simulink model "rfsoc4x2_ospfb_128"  (R2021a)
settings: Solver=VariableStepAuto  StartTime=0.0  StopTime=2048  RelTol=1e-3
undefined symbols (not defined in the file): pfb_coeff_gen_calc
libraries: xbsIndex_r4 x37092, casper_library_delays x737, casper_library_misc x68, xps_library x1
(part 146 of 339)

== system rfsoc4x2_ospfb_128/fft2/fft_unscrambler/debus4 ==
  bus_in : Inport
  reinterpret1 : xbsIndex_r4/Reinterpret  force_arith_type=on  arith_type=Unsigned  force_bin_pt=on  bin_pt=0  block_type=reinterpret
  slice1 : xbsIndex_r4/Slice  nbits=36  boolean_output=off  mode=Upper Bit Location + Width  bit1=0  base1=MSB of Input  bit0=0  base0=LSB of Input  dbl_ovrd=off  block_type=slice
  msb_lsb_out1 : Outport
  wires:
  reinterpret1/1 -> msb_lsb_out1/1
  slice1/1 -> reinterpret1/1
  bus_in/1 -> slice1/1

== system rfsoc4x2_ospfb_128/fft2/fft_unscrambler/debus5 ==
  bus_in : Inport
  reinterpret1 : xbsIndex_r4/Reinterpret  force_arith_type=on  arith_type=Unsigned  force_bin_pt=on  bin_pt=0  block_type=reinterpret
  slice1 : xbsIndex_r4/Slice  nbits=36  boolean_output=off  mode=Upper Bit Location + Width  bit1=0  base1=MSB of Input  bit0=0  base0=LSB of Input  dbl_ovrd=off  block_type=slice
  msb_lsb_out1 : Outport
  wires:
  reinterpret1/1 -> msb_lsb_out1/1
  slice1/1 -> reinterpret1/1
  bus_in/1 -> slice1/1

== system rfsoc4x2_ospfb_128/fft2/fft_unscrambler/debus6 ==
  bus_in : Inport
  reinterpret1 : xbsIndex_r4/Reinterpret  force_arith_type=on  arith_type=Unsigned  force_bin_pt=on  bin_pt=0  block_type=reinterpret
  slice1 : xbsIndex_r4/Slice  nbits=36  boolean_output=off  mode=Upper Bit Location + Width  bit1=0  base1=MSB of Input  bit0=0  base0=LSB of Input  dbl_ovrd=off  block_type=slice
  msb_lsb_out1 : Outport
  wires:
  reinterpret1/1 -> msb_lsb_out1/1
  slice1/1 -> reinterpret1/1
  bus_in/1 -> slice1/1

== system rfsoc4x2_ospfb_128/fft2/fft_unscrambler/debus7 ==
  bus_in : Inport
  reinterpret1 : xbsIndex_r4/Reinterpret  force_arith_type=on  arith_type=Unsigned  force_bin_pt=on  bin_pt=0  block_type=reinterpret
  slice1 : xbsIndex_r4/Slice  nbits=36  boolean_output=off  mode=Upper Bit Location + Width  bit1=0  base1=MSB of Input  bit0=0  base0=LSB of Input  dbl_ovrd=off  block_type=slice
  msb_lsb_out1 : Outport
  wires:
  reinterpret1/1 -> msb_lsb_out1/1
  slice1/1 -> reinterpret1/1
  bus_in/1 -> slice1/1

== system rfsoc4x2_ospfb_128/fft2/fft_unscrambler/reorder ==
  sync : Inport
  en : Inport  Port=2
  din0 : Inport  Port=3
  din1 : Inport  Port=4
  din2 : Inport  Port=5
  din3 : Inport  Port=6
  din4 : Inport  Port=7
  din5 : Inport  Port=8
  din6 : Inport  Port=9
  din7 : Inport  Port=10
  Counter : xbsIndex_r4/Counter  cnt_type=Free Running  cnt_to=Inf  operation=Up  start_count=0  cnt_by_val=1  arith_type=Unsigned  n_bits=7  bin_pt=0  load_pin=off  rst=on  en=on  explicit_period=on  period=1  use_behavioral_HDL=on  implementation=Fabric  dbl_ovrd=off  block_type=counter
  Mux : xbsIndex_r4/Mux  inputs=2  en=off  latency=1  precision=Full  arith_type=Unsigned  n_bits=16  bin_pt=14  quantization=Truncate  overflow=Wrap  dbl_ovrd=off  block_type=mux
  Slice1 : xbsIndex_r4/Slice  nbits=1  boolean_output=off  mode=Upper Bit Location + Width  bit1=0  base1=MSB of Input  bit0=0  base0=LSB of Input  dbl_ovrd=off  block_type=slice
  Slice2 : xbsIndex_r4/Slice  nbits=6  boolean_output=off  mode=Lower Bit Location + Width  bit1=0  base1=MSB of Input  bit0=0  base0=LSB of Input  dbl_ovrd=off  block_type=slice
  addr_expand : Subsystem  AncestorBlock=casper_library_flow_control/bus_expand  mask(bus_expand){mode=divisions of equal size, outputNum=8, outputWidth=6, outputBinaryPt=0, outputArithmeticType=0, show_format=off, outputToWorkspace=off, variablePrefix=out, outputToModelAsWell=on}
      mask prompts: outputNum "Number of outputs:"; outputWidth "Output width:"; outputBinaryPt "Output binary point position:"; outputArithmeticType "Output arithmetic type (ufix=0, fix=1, bool=2):"; show_format "Print format string?"; outputToWorkspace "Output to workspace?"; variablePrefix "Variable name prefix:"; outputToModelAsWell "Output to model as well?"
      mask help:
      | Expands a 'bus' made using a bus_create or Xilinx
      | concat block.
      | The input will be divided into the specified number
      | of outputs with the specified arithmetic types.
      | Divisions are made from most significant bit.
      mask init: same as rfsoc4x2_ospfb_128/bus_expand1
      settings: AttributesFormatString=8 outputs
      mask TypeOptions mode: divisions of equal size | divisions of arbitrary size
      mask Callback mode: %bus_expand_callback();
      mask Callback outputWidth: %bus_expand_callback();
      mask Callback outputToWorkspace: %bus_expand_callback();
  addr_replicate : Subsystem  AncestorBlock=casper_library_bus/bus_replicate  mask(bus_replicate){replication=8, csp_latency=3, misc=off, implementation=core}
      mask prompts: replication "replication factor"; csp_latency "latency"; misc "misc support"; implementation "delay implementation"
      mask help: Output bus formed by replicating input bus a number of times
      mask init:
      | bus_replicate_init(gcb, ...
      |     'replication', replication, ...
      |     'csp_latency', csp_latency, ...
      |     'implementation', implementation, ...
      |     'misc', misc);
      mask TypeOptions implementation: core | behavioral
  buf0 : Subsystem  AncestorBlock=casper_library_bus/bus_single_port_ram  mask(bus_single_port_ram){n_bits=[[repmat(64, 1, 0)], 36], bin_pts=[zeros(1, 1)], init_vector=[zeros(64,1)], max_fanout=1, mem_type=Block RAM, bram_optimization=Speed, async=off, misc=off, bram_latency=2, fan_latency=0, addr_register=on, addr_implementation=core, din_register=on, din_implementation=behavioral, we_register=on, we_implementation=core, en_register=off, en_implementation=behavioral}
      mask prompts: n_bits "data word bit widths"; bin_pts "data word binary points"; init_vector "initial value vector"; max_fanout "limit fanout to ?"; mem_type "memory type"; bram_optimization "memory optimization"; async "asynchronous"; misc "misc support"; bram_latency "bram latency"; fan_latency "input register latency"; addr_register "addr input register"; addr_implementation "addr register implementation"; din_register "din input register"; din_implementation "din register implementation"; we_register "we input register"; we_implementation "we register implementation"; en_register "en input register"; en_implementation "en register implementation"
      mask help: RAM for a bus allowing fanout control
      mask init:
      | bus_single_port_ram_init(gcb, ...
      |     'n_bits', n_bits, ...
      |     'bin_pts', bin_pts, ...
      |     'init_vector', init_vector, ...
      |     'max_fanout', max_fanout, ...
      |     'mem_type', mem_type, ...
      |     'bram_optimization', bram_optimization, ...
      |     'async', async, ...
      |     'misc', misc, ...
      |     'bram_latency', bram_latency, ...
      |     'fan_latency', fan_latency, ...
      |     'addr_register', addr_register, ...
      |     'addr_implementation', addr_implementation, ...
      |     'din_register', din_register, ...
      |     'din_implementation', din_implementation, ...
      |     'we_register', we_register, ...
      |     'we_implementation', we_implementation, ...
      |     'en_register', en_register, ...
      |     'en_implementation', en_implementation);
      mask TypeOptions mem_type: Distributed memory | Block RAM
      mask TypeOptions bram_optimization: Area | Speed
      mask TypeOptions addr_implementation: core | behavioral
      mask TypeOptions din_implementation: core | behavioral
      mask TypeOptions we_implementation: core | behavioral
      mask TypeOptions en_implementation: core | behavioral
  buf1 : Subsystem  AncestorBlock=casper_library_bus/bus_single_port_ram  mask(bus_single_port_ram){n_bits=[[repmat(64, 1, 0)], 36], bin_pts=[zeros(1, 1)], init_vector=[zeros(64,1)], max_fanout=1, mem_type=Block RAM, bram_optimization=Speed, async=off, misc=off, bram_latency=2, fan_latency=0, addr_register=on, addr_implementation=core, din_register=on, din_implementation=behavioral, we_register=on, we_implementation=core, en_register=off, en_implementation=behavioral}
      mask prompts: n_bits "data word bit widths"; bin_pts "data word binary points"; init_vector "initial value vector"; max_fanout "limit fanout to ?"; mem_type "memory type"; bram_optimization "memory optimization"; async "asynchronous"; misc "misc support"; bram_latency "bram latency"; fan_latency "input register latency"; addr_register "addr input register"; addr_implementation "addr register implementation"; din_register "din input register"; din_implementation "din register implementation"; we_register "we input register"; we_implementation "we register implementation"; en_register "en input register"; en_implementation "en register implementation"
      mask help: RAM for a bus allowing fanout control
      mask init: same as rfsoc4x2_ospfb_128/fft2/fft_unscrambler/reorder/buf0
      mask TypeOptions mem_type: Distributed memory | Block RAM
      mask TypeOptions bram_optimization: Area | Speed
      mask TypeOptions addr_implementation: core | behavioral
      mask TypeOptions din_implementation: core | behavioral
      mask TypeOptions we_implementation: core | behavioral
      mask TypeOptions en_implementation: core | behavioral
  buf2 : Subsystem  AncestorBlock=casper_library_bus/bus_single_port_ram  mask(bus_single_port_ram){n_bits=[[repmat(64, 1, 0)], 36], bin_pts=[zeros(1, 1)], init_vector=[zeros(64,1)], max_fanout=1, mem_type=Block RAM, bram_optimization=Speed, async=off, misc=off, bram_latency=2, fan_latency=0, addr_register=on, addr_implementation=core, din_register=on, din_implementation=behavioral, we_register=on, we_implementation=core, en_register=off, en_implementation=behavioral}
      mask prompts: n_bits "data word bit widths"; bin_pts "data word binary points"; init_vector "initial value vector"; max_fanout "limit fanout to ?"; mem_type "memory type"; bram_optimization "memory optimization"; async "asynchronous"; misc "misc support"; bram_latency "bram latency"; fan_latency "input register latency"; addr_register "addr input register"; addr_implementation "addr register implementation"; din_register "din input register"; din_implementation "din register implementation"; we_register "we input register"; we_implementation "we register implementation"; en_register "en input register"; en_implementation "en register implementation"
      mask help: RAM for a bus allowing fanout control
      mask init: same as rfsoc4x2_ospfb_128/fft2/fft_unscrambler/reorder/buf0
      mask TypeOptions mem_type: Distributed memory | Block RAM
      mask TypeOptions bram_optimization: Area | Speed
      mask TypeOptions addr_implementation: core | behavioral
      mask TypeOptions din_implementation: core | behavioral
      mask TypeOptions we_implementation: core | behavioral
      mask TypeOptions en_implementation: core | behavioral
  buf3 : Subsystem  AncestorBlock=casper_library_bus/bus_single_port_ram  mask(bus_single_port_ram){n_bits=[[repmat(64, 1, 0)], 36], bin_pts=[zeros(1, 1)], init_vector=[zeros(64,1)], max_fanout=1, mem_type=Block RAM, bram_optimization=Speed, async=off, misc=off, bram_latency=2, fan_latency=0, addr_register=on, addr_implementation=core, din_register=on, din_implementation=behavioral, we_register=on, we_implementation=core, en_register=off, en_implementation=behavioral}
      mask prompts: n_bits "data word bit widths"; bin_pts "data word binary points"; init_vector "initial value vector"; max_fanout "limit fanout to ?"; mem_type "memory type"; bram_optimization "memory optimization"; async "asynchronous"; misc "misc support"; bram_latency "bram latency"; fan_latency "input register latency"; addr_register "addr input register"; addr_implementation "addr register implementation"; din_register "din input register"; din_implementation "din register implementation"; we_register "we input register"; we_implementation "we register implementation"; en_register "en input register"; en_implementation "en register implementation"
      mask help: RAM for a bus allowing fanout control
      mask init: same as rfsoc4x2_ospfb_128/fft2/fft_unscrambler/reorder/buf0
      mask TypeOptions mem_type: Distributed memory | Block RAM
      mask TypeOptions bram_optimization: Area | Speed
      mask TypeOptions addr_implementation: core | behavioral
      mask TypeOptions din_implementation: core | behavioral
      mask TypeOptions we_implementation: core | behavioral
      mask TypeOptions en_implementation: core | behavioral
  buf4 : Subsystem  AncestorBlock=casper_library_bus/bus_single_port_ram  mask(bus_single_port_ram){n_bits=[[repmat(64, 1, 0)], 36], bin_pts=[zeros(1, 1)], init_vector=[zeros(64,1)], max_fanout=1, mem_type=Block RAM, bram_optimization=Speed, async=off, misc=off, bram_latency=2, fan_latency=0, addr_register=on, addr_implementation=core, din_register=on, din_implementation=behavioral, we_register=on, we_implementation=core, en_register=off, en_implementation=behavioral}
      mask prompts: n_bits "data word bit widths"; bin_pts "data word binary points"; init_vector "initial value vector"; max_fanout "limit fanout to ?"; mem_type "memory type"; bram_optimization "memory optimization"; async "asynchronous"; misc "misc support"; bram_latency "bram latency"; fan_latency "input register latency"; addr_register "addr input register"; addr_implementation "addr register implementation"; din_register "din input register"; din_implementation "din register implementation"; we_register "we input register"; we_implementation "we register implementation"; en_register "en input register"; en_implementation "en register implementation"
      mask help: RAM for a bus allowing fanout control
      mask init: same as rfsoc4x2_ospfb_128/fft2/fft_unscrambler/reorder/buf0
      mask TypeOptions mem_type: Distributed memory | Block RAM
      mask TypeOptions bram_optimization: Area | Speed
      mask TypeOptions addr_implementation: core | behavioral
      mask TypeOptions din_implementation: core | behavioral
      mask TypeOptions we_implementation: core | behavioral
      mask TypeOptions en_implementation: core | behavioral
  buf5 : Subsystem  AncestorBlock=casper_library_bus/bus_single_port_ram  mask(bus_single_port_ram){n_bits=[[repmat(64, 1, 0)], 36], bin_pts=[zeros(1, 1)], init_vector=[zeros(64,1)], max_fanout=1, mem_type=Block RAM, bram_optimization=Speed, async=off, misc=off, bram_latency=2, fan_latency=0, addr_register=on, addr_implementation=core, din_register=on, din_implementation=behavioral, we_register=on, we_implementation=core, en_register=off, en_implementation=behavioral}
      mask prompts: n_bits "data word bit widths"; bin_pts "data word binary points"; init_vector "initial value vector"; max_fanout "limit fanout to ?"; mem_type "memory type"; bram_optimization "memory optimization"; async "asynchronous"; misc "misc support"; bram_latency "bram latency"; fan_latency "input register latency"; addr_register "addr input register"; addr_implementation "addr register implementation"; din_register "din input register"; din_implementation "din register implementation"; we_register "we input register"; we_implementation "we register implementation"; en_register "en input register"; en_implementation "en register implementation"
      mask help: RAM for a bus allowing fanout control
      mask init: same as rfsoc4x2_ospfb_128/fft2/fft_unscrambler/reorder/buf0
      mask TypeOptions mem_type: Distributed memory | Block RAM
      mask TypeOptions bram_optimization: Area | Speed
      mask TypeOptions addr_implementation: core | behavioral
      mask TypeOptions din_implementation: core | behavioral
      mask TypeOptions we_implementation: core | behavioral
      mask TypeOptions en_implementation: core | behavioral
  buf6 : Subsystem  AncestorBlock=casper_library_bus/bus_single_port_ram  mask(bus_single_port_ram){n_bits=[[repmat(64, 1, 0)], 36], bin_pts=[zeros(1, 1)], init_vector=[zeros(64,1)], max_fanout=1, mem_type=Block RAM, bram_optimization=Speed, async=off, misc=off, bram_latency=2, fan_latency=0, addr_register=on, addr_implementation=core, din_register=on, din_implementation=behavioral, we_register=on, we_implementation=core, en_register=off, en_implementation=behavioral}
      mask prompts: n_bits "data word bit widths"; bin_pts "data word binary points"; init_vector "initial value vector"; max_fanout "limit fanout to ?"; mem_type "memory type"; bram_optimization "memory optimization"; async "asynchronous"; misc "misc support"; bram_latency "bram latency"; fan_latency "input register latency"; addr_register "addr input register"; addr_implementation "addr register implementation"; din_register "din input register"; din_implementation "din register implementation"; we_register "we input register"; we_implementation "we register implementation"; en_register "en input register"; en_implementation "en register implementation"
      mask help: RAM for a bus allowing fanout control
      mask init: same as rfsoc4x2_ospfb_128/fft2/fft_unscrambler/reorder/buf0
      mask TypeOptions mem_type: Distributed memory | Block RAM
      mask TypeOptions bram_optimization: Area | Speed
      mask TypeOptions addr_implementation: core | behavioral
      mask TypeOptions din_implementation: core | behavioral
      mask TypeOptions we_implementation: core | behavioral
      mask TypeOptions en_implementation: core | behavioral
  buf7 : Subsystem  AncestorBlock=casper_library_bus/bus_single_port_ram  mask(bus_single_port_ram){n_bits=[[repmat(64, 1, 0)], 36], bin_pts=[zeros(1, 1)], init_vector=[zeros(64,1)], max_fanout=1, mem_type=Block RAM, bram_optimization=Speed, async=off, misc=off, bram_latency=2, fan_latency=0, addr_register=on, addr_implementation=core, din_register=on, din_implementation=behavioral, we_register=on, we_implementation=core, en_register=off, en_implementation=behavioral}
      mask prompts: n_bits "data word bit widths"; bin_pts "data word binary points"; init_vector "initial value vector"; max_fanout "limit fanout to ?"; mem_type "memory type"; bram_optimization "memory optimization"; async "asynchronous"; misc "misc support"; bram_latency "bram latency"; fan_latency "input register latency"; addr_register "addr input register"; addr_implementation "addr register implementation"; din_register "din input register"; din_implementation "din register implementation"; we_register "we input register"; we_implementation "we register implementation"; en_register "en input register"; en_implementation "en register implementation"
      mask help: RAM for a bus allowing fanout control
      mask init: same as rfsoc4x2_ospfb_128/fft2/fft_unscrambler/reorder/buf0
      mask TypeOptions mem_type: Distributed memory | Block RAM
      mask TypeOptions bram_optimization: Area | Speed
      mask TypeOptions addr_implementation: core | behavioral
      mask TypeOptions din_implementation: core | behavioral
      mask TypeOptions we_implementation: core | behavioral
      mask TypeOptions en_implementation: core | behavioral
  delay_d0 : xbsIndex_r4/Delay  rst=off  infoeditControl=Selection of Reset will increase slice count due to use of real FFs and instead of SRLs  en=off  latency=2  reg_retiming=on  dbl_ovrd=off  block_type=delay
  delay_din{0..7} (8 alike) : xbsIndex_r4/Delay  rst=off  infoeditControl=Selection of Reset will increase slice count due to use of real FFs and instead of SRLs  en=off  latency=6  reg_retiming=on  dbl_ovrd=off  block_type=delay
  delay_map1 : xbsIndex_r4/Delay  rst=off  infoeditControl=Selection of Reset will increase slice count due to use of real FFs and instead of SRLs  en=off  latency=0  reg_retiming=on  dbl_ovrd=off  block_type=delay
  delay_sel : xbsIndex_r4/Delay  rst=off  infoeditControl=Selection of Reset will increase slice count due to use of real FFs and instead of SRLs  en=off  latency=2  reg_retiming=on  dbl_ovrd=off  block_type=delay
  delay_valid : xbsIndex_r4/Delay  rst=off  infoeditControl=Selection of Reset will increase slice count due to use of real FFs and instead of SRLs  en=off  latency=2  reg_retiming=on  dbl_ovrd=off  block_type=delay
  delay_we0 : xbsIndex_r4/Delay  rst=off  infoeditControl=Selection of Reset will increase slice count due to use of real FFs and instead of SRLs  en=off  latency=6  reg_retiming=on  dbl_ovrd=off  block_type=delay
  delay_we1 : xbsIndex_r4/Delay  rst=off  infoeditControl=Selection of Reset will increase slice count due to use of real FFs and instead of SRLs  en=off  latency=6  reg_retiming=on  dbl_ovrd=off  block_type=delay
  delay_we2 : xbsIndex_r4/Delay  rst=off  infoeditControl=Selection of Reset will increase slice count due to use of real FFs and instead of SRLs  en=off  latency=3  reg_retiming=on  dbl_ovrd=off  block_type=delay
  map1 : xbsIndex_r4/ROM  depth=64  initVector=map  distributed_mem=Block RAM  rst=off  init_reg=0  en=off  latency=2  gui_display_data_type=Fixed-point  arith_type=Unsigned  n_bits=6  bin_pt=0  preci_type=Single  exp_width=8  frac_width=24  optimize=Speed  use_rpm=on  dbl_ovrd=off  simulation_type=fast_sim  block_type=sprom
  or : xbsIndex_r4/Logical  logical_function=OR  inputs=2  en=off  latency=0  precision=Full  arith_type=Unsigned  n_bits=16  bin_pt=0  align_bp=on  dbl_ovrd=off  block_type=logical
  post_sync_delay : xbsIndex_r4/Delay  rst=off  infoeditControl=Selection of Reset will increase slice count due to use of real FFs and instead of SRLs  en=off  latency=2  reg_retiming=on  dbl_ovrd=off  block_type=delay
  pre_sync_delay : xbsIndex_r4/Delay  rst=off  infoeditControl=Selection of Reset will increase slice count due to use of real FFs and instead of SRLs  en=off  latency=6  reg_retiming=on  dbl_ovrd=off  block_type=delay
  sync_delay_en : casper_library_delays/sync_delay_en  DelayLen=64
      settings: SourceProductName=CASPER DSP Blockset
  we_expand : Subsystem  AncestorBlock=casper_library_flow_control/bus_expand  mask(bus_expand){mode=divisions of equal size, outputNum=8, outputWidth=1, outputBinaryPt=0, outputArithmeticType=2, show_format=off, outputToWorkspace=off, variablePrefix=out, outputToModelAsWell=on}
      mask prompts: outputNum "Number of outputs:"; outputWidth "Output width:"; outputBinaryPt "Output binary point position:"; outputArithmeticType "Output arithmetic type (ufix=0, fix=1, bool=2):"; show_format "Print format string?"; outputToWorkspace "Output to workspace?"; variablePrefix "Variable name prefix:"; outputToModelAsWell "Output to model as well?"
      mask help:
      | Expands a 'bus' made using a bus_create or Xilinx
      | concat block.
      | The input will be divided into the specified number
      | of outputs with the specified arithmetic types.
      | Divisions are made from most significant bit.
      mask init: same as rfsoc4x2_ospfb_128/bus_expand1
      settings: AttributesFormatString=8 outputs
      mask TypeOptions mode: divisions of equal size | divisions of arbitrary size
      mask Callback mode: %bus_expand_callback();
      mask Callback outputWidth: %bus_expand_callback();
      mask Callback outputToWorkspace: %bus_expand_callback();
  we_replicate : Subsystem  AncestorBlock=casper_library_bus/bus_replicate  mask(bus_replicate){replication=8, csp_latency=3, misc=off, implementation=core}
      mask prompts: replication "replication factor"; csp_latency "latency"; misc "misc support"; implementation "delay implementation"
      mask help: Output bus formed by replicating input bus a number of times
      mask init:
      | bus_replicate_init(gcb, ...
      |     'replication', replication, ...
      |     'csp_latency', csp_latency, ...
      |     'implementation', implementation, ...
      |     'misc', misc);
      mask TypeOptions implementation: core | behavioral
  sync_out : Outport
  valid : Outport  Port=2
  dout0 : Outport  Port=3
  dout1 : Outport  Port=4
  dout2 : Outport  Port=5
  dout3 : Outport  Port=6
  dout4 : Outport  Port=7
  dout5 : Outport  Port=8
  dout6 : Outport  Port=9
  dout7 : Outport  Port=10
  wires:
  delay_map1/1 -> Mux/3
  map1/1 -> delay_map1/1
  Mux/1 -> addr_replicate/1(in)
  delay_d0/1 -> Mux/2
  delay_sel/1 -> Mux/1
  Slice1/1 -> delay_sel/1
  buf7/1(dout) -> dout7/1
  delay_din7/1 -> buf7/2(din)
  addr_expand/8(lsb_out1) -> buf7/1(addr)
  we_expand/8(lsb_out1) -> buf7/3(we)
  buf6/1(dout) -> dout6/1
  delay_din6/1 -> buf6/2(din)
  addr_expand/7(out2) -> buf6/1(addr)
  we_expand/7(out2) -> buf6/3(we)
  buf5/1(dout) -> dout5/1
  delay_din5/1 -> buf5/2(din)
  addr_expand/6(out3) -> buf5/1(addr)
  we_expand/6(out3) -> buf5/3(we)
  buf4/1(dout) -> dout4/1
  delay_din4/1 -> buf4/2(din)
  addr_expand/5(out4) -> buf4/1(addr)
  we_expand/5(out4) -> buf4/3(we)
  buf3/1(dout) -> dout3/1
  delay_din3/1 -> buf3/2(din)
  addr_expand/4(out5) -> buf3/1(addr)
  we_expand/4(out5) -> buf3/3(we)
  buf2/1(dout) -> dout2/1
  delay_din2/1 -> buf2/2(din)
  addr_expand/3(out6) -> buf2/1(addr)
  we_expand/3(out6) -> buf2/3(we)
  buf1/1(dout) -> dout1/1
  delay_din1/1 -> buf1/2(din)
  addr_expand/2(out7) -> buf1/1(addr)
  we_expand/2(out7) -> buf1/3(we)
  buf0/1(dout) -> dout0/1
  delay_din0/1 -> buf0/2(din)
  addr_expand/1(msb_out8) -> buf0/1(addr)
  we_expand/1(msb_out8) -> buf0/3(we)
  addr_replicate/1(out) -> addr_expand/1(bus_in)
  Slice2/1 -> map1/1, delay_d0/1
  Counter/1 -> Slice1/1, Slice2/1
  din7/1 -> delay_din7/1
  din6/1 -> delay_din6/1
  din5/1 -> delay_din5/1
  din4/1 -> delay_din4/1
  din3/1 -> delay_din3/1
  din2/1 -> delay_din2/1
  din1/1 -> delay_din1/1
  din0/1 -> delay_din0/1
  post_sync_delay/1 -> sync_out/1
  sync_delay_en/1 -> post_sync_delay/1
  or/1 -> sync_delay_en/2
  pre_sync_delay/1 -> sync_delay_en/1, or/1
  delay_we0/1 -> or/2
  sync/1 -> Counter/1, pre_sync_delay/1
  we_replicate/1(out) -> we_expand/1(bus_in)
  delay_we2/1 -> we_replicate/1(in)
  delay_valid/1 -> valid/1
  delay_we1/1 -> delay_valid/1
  en/1 -> Counter/2, delay_we2/1, delay_we1/1, delay_we0/1

== system rfsoc4x2_ospfb_128/fft2/fft_unscrambler/square_transposer ==
  sync : Inport
  in0 : Inport  Port=2
  in1 : Inport  Port=3
  in2 : Inport  Port=4
  in3 : Inport  Port=5
  in4 : Inport  Port=6
  in5 : Inport  Port=7
  in6 : Inport  Port=8
  in7 : Inport  Port=9
  barrel_switcher : Subsystem  AncestorBlock=casper_library_reorder/barrel_switcher  mask(barrel_switcher){n_inputs=3, async=off}
      mask prompts: n_inputs "Number of Inputs: (2^?)"; async "Asynchronous operation"
      mask help:
      | Shifts input to right by amount specified on sel,
      | wrapping around into higher order bits.
      mask init:
      | barrel_switcher_init(gcb,...
      |     'n_inputs', n_inputs, ...
      |     'async', async);
      mask Help: eval('xlWeb(''http://casper.berkeley.edu/wiki/Barrel_switcher'')')
  counter : xbsIndex_r4/Counter  cnt_type=Free Running  cnt_to=Inf  operation=Down  start_count=0  cnt_by_val=1  arith_type=Unsigned  n_bits=n_inputs  bin_pt=0  load_pin=off  rst=on  en=off  explicit_period=on  period=1  use_behavioral_HDL=off  implementation=Fabric  dbl_ovrd=off  block_type=counter
  db0 : Subsystem  AncestorBlock=casper_library_delays/delay_slr  mask(delay_slr){DelayLen=7, async=off}
      mask prompts: DelayLen "Delay by:"; async "asynchronous operation"
      mask help: A delay block that uses slices (SLR16s) for its storage.
      mask init:
      | delay_slr_init(gcb, ...
      |     'DelayLen', DelayLen, ...
      |     'async', async);
  db1 : Subsystem  AncestorBlock=casper_library_delays/delay_slr  mask(delay_slr){DelayLen=6, async=off}
      mask prompts: DelayLen "Delay by:"; async "asynchronous operation"
      mask help: A delay block that uses slices (SLR16s) for its storage.
      mask init:
      | delay_slr_init(gcb, ...
      |     'DelayLen', DelayLen, ...
      |     'async', async);
  db2 : Subsystem  AncestorBlock=casper_library_delays/delay_slr  mask(delay_slr){DelayLen=5, async=off}
      mask prompts: DelayLen "Delay by:"; async "asynchronous operation"
      mask help: A delay block that uses slices (SLR16s) for its storage.
      mask init:
      | delay_slr_init(gcb, ...
      |     'DelayLen', DelayLen, ...
      |     'async', async);
  db3 : Subsystem  AncestorBlock=casper_library_delays/delay_slr  mask(delay_slr){DelayLen=4, async=off}
      mask prompts: DelayLen "Delay by:"; async "asynchronous operation"
      mask help: A delay block that uses slices (SLR16s) for its storage.
      mask init:
      | delay_slr_init(gcb, ...
      |     'DelayLen', DelayLen, ...
      |     'async', async);
  db4 : Subsystem  AncestorBlock=casper_library_delays/delay_slr  mask(delay_slr){DelayLen=3, async=off}
      mask prompts: DelayLen "Delay by:"; async "asynchronous operation"
      mask help: A delay block that uses slices (SLR16s) for its storage.
      mask init:
      | delay_slr_init(gcb, ...
      |     'DelayLen', DelayLen, ...
      |     'async', async);
  db5 : Subsystem  AncestorBlock=casper_library_delays/delay_slr  mask(delay_slr){DelayLen=2, async=off}
      mask prompts: DelayLen "Delay by:"; async "asynchronous operation"
      mask help: A delay block that uses slices (SLR16s) for its storage.
      mask init:
      | delay_slr_init(gcb, ...
      |     'DelayLen', DelayLen, ...
      |     'async', async);
  db6 : Subsystem  AncestorBlock=casper_library_delays/delay_slr  mask(delay_slr){DelayLen=1, async=off}
      mask prompts: DelayLen "Delay by:"; async "asynchronous operation"
      mask help: A delay block that uses slices (SLR16s) for its storage.
      mask init:
      | delay_slr_init(gcb, ...
      |     'DelayLen', DelayLen, ...
      |     'async', async);
  df1 : Subsystem  AncestorBlock=casper_library_delays/delay_slr  mask(delay_slr){DelayLen=1, async=off}
      mask prompts: DelayLen "Delay by:"; async "asynchronous operation"
      mask help: A delay block that uses slices (SLR16s) for its storage.
      mask init:
      | delay_slr_init(gcb, ...
      |     'DelayLen', DelayLen, ...
      |     'async', async);
  df2 : Subsystem  AncestorBlock=casper_library_delays/delay_slr  mask(delay_slr){DelayLen=2, async=off}
      mask prompts: DelayLen "Delay by:"; async "asynchronous operation"
      mask help: A delay block that uses slices (SLR16s) for its storage.
      mask init:
      | delay_slr_init(gcb, ...
      |     'DelayLen', DelayLen, ...
      |     'async', async);
  df3 : Subsystem  AncestorBlock=casper_library_delays/delay_slr  mask(delay_slr){DelayLen=3, async=off}
      mask prompts: DelayLen "Delay by:"; async "asynchronous operation"
      mask help: A delay block that uses slices (SLR16s) for its storage.
      mask init:
      | delay_slr_init(gcb, ...
      |     'DelayLen', DelayLen, ...
      |     'async', async);
  df4 : Subsystem  AncestorBlock=casper_library_delays/delay_slr  mask(delay_slr){DelayLen=4, async=off}
      mask prompts: DelayLen "Delay by:"; async "asynchronous operation"
      mask help: A delay block that uses slices (SLR16s) for its storage.
      mask init:
      | delay_slr_init(gcb, ...
      |     'DelayLen', DelayLen, ...
      |     'async', async);
  df5 : Subsystem  AncestorBlock=casper_library_delays/delay_slr  mask(delay_slr){DelayLen=5, async=off}
      mask prompts: DelayLen "Delay by:"; async "asynchronous operation"
      mask help: A delay block that uses slices (SLR16s) for its storage.
      mask init:
      | delay_slr_init(gcb, ...
      |     'DelayLen', DelayLen, ...
      |     'async', async);
  df6 : Subsystem  AncestorBlock=casper_library_delays/delay_slr  mask(delay_slr){DelayLen=6, async=off}
      mask prompts: DelayLen "Delay by:"; async "asynchronous operation"
      mask help: A delay block that uses slices (SLR16s) for its storage.
      mask init:
      | delay_slr_init(gcb, ...
      |     'DelayLen', DelayLen, ...
      |     'async', async);
  df7 : Subsystem  AncestorBlock=casper_library_delays/delay_slr  mask(delay_slr){DelayLen=7, async=off}
      mask prompts: DelayLen "Delay by:"; async "asynchronous operation"
      mask help: A delay block that uses slices (SLR16s) for its storage.
      mask init:
      | delay_slr_init(gcb, ...
      |     'DelayLen', DelayLen, ...
      |     'async', async);
  dsync : Subsystem  AncestorBlock=casper_library_delays/delay_slr  mask(delay_slr){DelayLen=7, async=off}
      mask prompts: DelayLen "Delay by:"; async "asynchronous operation"
      mask help: A delay block that uses slices (SLR16s) for its storage.
      mask init:
      | delay_slr_init(gcb, ...
      |     'DelayLen', DelayLen, ...
      |     'async', async);
  sync_out : Outport
  out0 : Outport  Port=2
  out1 : Outport  Port=3
  out2 : Outport  Port=4
  out3 : Outport  Port=5
  out4 : Outport  Port=6
  out5 : Outport  Port=7
  out6 : Outport  Port=8
  out7 : Outport  Port=9
  wires:
  barrel_switcher/9(Out8) -> out7/1
  df7/1(dout) -> barrel_switcher/4(In2)
  in7/1 -> df7/1(din)
  db6/1(dout) -> out6/1
  barrel_switcher/8(Out7) -> db6/1(din)
  df6/1(dout) -> barrel_switcher/5(In3)
  in6/1 -> df6/1(din)
  db5/1(dout) -> out5/1
  barrel_switcher/7(Out6) -> db5/1(din)
  df5/1(dout) -> barrel_switcher/6(In4)
  in5/1 -> df5/1(din)
  db4/1(dout) -> out4/1
  barrel_switcher/6(Out5) -> db4/1(din)
  df4/1(dout) -> barrel_switcher/7(In5)
  in4/1 -> df4/1(din)
  db3/1(dout) -> out3/1
  barrel_switcher/5(Out4) -> db3/1(din)
  df3/1(dout) -> barrel_switcher/8(In6)
  in3/1 -> df3/1(din)
  db2/1(dout) -> out2/1
  barrel_switcher/4(Out3) -> db2/1(din)
  df2/1(dout) -> barrel_switcher/9(In7)
  in2/1 -> df2/1(din)
  db1/1(dout) -> out1/1
  barrel_switcher/3(Out2) -> db1/1(din)
  df1/1(dout) -> barrel_switcher/10(In8)
  in1/1 -> df1/1(din)
  db0/1(dout) -> out0/1
  barrel_switcher/2(Out1) -> db0/1(din)
  in0/1 -> barrel_switcher/3(In1)
  barrel_switcher/1(sync_out) -> dsync/1(din)
  counter/1 -> barrel_switcher/1(sel)
  dsync/1(dout) -> sync_out/1
  sync/1 -> barrel_switcher/2(sync_in), counter/1
